simulink model "Dll_Control_AFO_V8_5_R2019b"  (R2019b)
settings: Solver=ode2  StartTime=0.0  StopTime=10  FixedStep=Ts  RelTol=1e-3
InitFcn:
  | modelDir=fileparts(get_param(bdroot,'FileName'));addpath(modelDir);rootDir=fileparts(modelDir);if isfolder(rootDir),addpath(rootDir);end;fmuDir=fullfile(rootDir,'fmu');if isfolder(fmuDir),addpath(fmuDir);end;if evalin('base','exist(''Wf0'',''var'')'),assignin('base','Wfb',evalin('base','Wf0'));end;
values from neighbouring files (symbols this model uses):
  A80 = 0.10573    [RunCtrlSysModelSHT.m]
  b11 = B(1,1)*1    [RunCtrlSysModelSHT.m]
  b21 = B(2,1)*1    [RunCtrlSysModelSHT.m]
  d31 = D(3,1)    [RunCtrlSysModelSHT.m]
  d41 = D(4,1)    [RunCtrlSysModelSHT.m]
  ExternalSecondaryAirEnabled = 0    [RunCtrlSysModelSHT.m]
  InitAir = zeros(50,1)    [RunCtrlSysModelSHT.m]
  Mkg0 = 0    [RunCtrlSysModelSHT.m]
  MkpDirectCommand = Mkp0    (= 999.278795578)    [RunCtrlSysModelSHT.m]
  MkpMax = 1200    [RunCtrlSysModelSHT.m]
  Ng0 = 38000    [RunCtrlSysModelSHT.m]
  NgMax = Ng0*1.05    (= 39900)    [RunCtrlSysModelSHT.m]
  Np0 = 20800    [RunCtrlSysModelSHT.m]
  NpDem = Np0    (= 20800)    [RunCtrlSysModelSHT.m]
  omega_u = 20    [RunCtrlSysModelSHT.m]
  power0 = 2176600    [RunCtrlSysModelSHT.m]
  RotorLoadCfg = struct(      'designNpRpm', Np0,      'designPowerW', power0,      'thetaZeroDeg', 0,      'thetaDesignDeg', 12,      'profileTorqueFraction', 0.15,      'thetaValidRangeDeg', [6, 14])    [RunCtrlSysModelSHT.m]
  RotorLoadInputMode = 'legacyPower'    [RunCtrlSysModelSHT.m]
  T45Max = 1400    [RunCtrlSysModelSHT.m]
  ThetaCommandDeg = RotorLoadCfg.thetaDesignDeg    [RunCtrlSysModelSHT.m]
  Ts = 0.025    [RunCtrlSysModelSHT.m]
  Wf0 = 0.151914044493225    (= 0.151914044493)    [RunCtrlSysModelSHT.m]
  WfMax = Wf0*2    (= 0.303828088986)    [RunCtrlSysModelSHT.m]
  WfMin = Wf0*0.01    (= 0.00151914044493)    [RunCtrlSysModelSHT.m]
  WfRateLim = 1.5    [RunCtrlSysModelSHT.m]
undefined symbols (not defined in the file or in its folder): sigbuilder_block, Wfb
libraries: simulink x10
(part 2 of 4)

== system Dll_Control_AFO_V8_5_R2019b/空气系统代理模型/G05_动力涡轮一级叶根进口 ==
  BoundaryTP24 : Inport  PortDimensions=24
  RotorSpeed_rpm : Inport  Port=2  PortDimensions=1
  GlobalParams7 : Inport  Port=3  PortDimensions=7
  EffectiveAreaScale : Selector  InputPortWidth=7  IndexOptions=Index vector (dialog)  Indices=1  OutputSizes=1
  SealCorrection : Selector  InputPortWidth=7  IndexOptions=Index vector (dialog)  Indices=7  OutputSizes=1
  可压缩节流孔口 : Subsystem  Description=Embedded ideal-gas compressible restrictor with critical pressure ratio. No external MATLAB runtime function.  mask{UpstreamBoundary=11, DownstreamBoundary=8}
      mask prompts: UpstreamBoundary "Upstream boundary index"; DownstreamBoundary "Downstream boundary index"
  导叶冷却 : Gain  Gain=0.90000000000000002
  旋转离心压升 : Subsystem  Description=Embedded centrifugal pressure rise: 0.5*kRot*rho*omega^2*(rOut^2-rIn^2).  mask{UpstreamBoundary=11, DownstreamBoundary=8}
      mask prompts: UpstreamBoundary "Upstream boundary index"; DownstreamBoundary "Downstream boundary index"
  流路可调参数 : Subsystem  Description=流路级可调物理参数（已内置在 SLX）。
  流量物理限幅 : Saturate  UpperLimit=2  LowerLimit=0
  盘腔热动态 : Subsystem  Description=Embedded discrete first-order lag with exact bypass when tau is zero.  mask{SampleTime_s=0.025000000000000001, InitialFlowValue=0.038254988453198698}
      mask prompts: SampleTime_s "Sample time [s]"; InitialFlowValue "Initial output [kg/s]"
  等效面积缩放 : Product  Inputs=**
  篦齿修正 : Product  Inputs=**
  辨识等效面积 : Subsystem  Description=辨识得到的等效面积律（内嵌 MATLAB Function）。
  G05_PT1_IN_ROOT_W_kgps : Outport
  wires:
  流量物理限幅/1 -> G05_PT1_IN_ROOT_W_kgps/1
  盘腔热动态/1(W_out) -> 流量物理限幅/1
  篦齿修正/1 -> 盘腔热动态/1(W_in)
  EffectiveAreaScale/1 -> 等效面积缩放/2
  SealCorrection/1 -> 篦齿修正/2
  导叶冷却/1 -> 篦齿修正/1
  旋转离心压升/1(W_out) -> 导叶冷却/1
  RotorSpeed_rpm/1 -> 旋转离心压升/3(RotorSpeed_rpm)
  可压缩节流孔口/1(W_kgps) -> 旋转离心压升/1(W_in)
  GlobalParams7/1 -> 可压缩节流孔口/3(GlobalParams7), 旋转离心压升/4(GlobalParams7)
  等效面积缩放/1 -> 可压缩节流孔口/2(EffectiveArea_m2)
  辨识等效面积/1(EffectiveArea_m2) -> 等效面积缩放/1
  BoundaryTP24/1 -> 可压缩节流孔口/1(BoundaryTP24), 旋转离心压升/2(BoundaryTP24), 辨识等效面积/1(BoundaryTP24)
  流路可调参数/1(RouteParams7) -> SealCorrection/1, 盘腔热动态/2(RouteParams7), 旋转离心压升/5(RouteParams7), EffectiveAreaScale/1

== system Dll_Control_AFO_V8_5_R2019b/空气系统代理模型/G06_动力涡轮一级叶根出口 ==
  BoundaryTP24 : Inport  PortDimensions=24
  RotorSpeed_rpm : Inport  Port=2  PortDimensions=1
  GlobalParams7 : Inport  Port=3  PortDimensions=7
  EffectiveAreaScale : Selector  InputPortWidth=7  IndexOptions=Index vector (dialog)  Indices=1  OutputSizes=1
  SealCorrection : Selector  InputPortWidth=7  IndexOptions=Index vector (dialog)  Indices=7  OutputSizes=1
  可压缩节流孔口 : Subsystem  Description=Embedded ideal-gas compressible restrictor with critical pressure ratio. No external MATLAB runtime function.  mask{UpstreamBoundary=11, DownstreamBoundary=5}
      mask prompts: UpstreamBoundary "Upstream boundary index"; DownstreamBoundary "Downstream boundary index"
  旋转离心压升 : Subsystem  Description=Embedded centrifugal pressure rise: 0.5*kRot*rho*omega^2*(rOut^2-rIn^2).  mask{UpstreamBoundary=11, DownstreamBoundary=5}
      mask prompts: UpstreamBoundary "Upstream boundary index"; DownstreamBoundary "Downstream boundary index"
  流路可调参数 : Subsystem  Description=流路级可调物理参数（已内置在 SLX）。
  流量物理限幅 : Saturate  UpperLimit=2  LowerLimit=0
  盘腔热动态 : Subsystem  Description=Embedded discrete first-order lag with exact bypass when tau is zero.  mask{SampleTime_s=0.025000000000000001, InitialFlowValue=0.0308724468218796}
      mask prompts: SampleTime_s "Sample time [s]"; InitialFlowValue "Initial output [kg/s]"
  等效面积缩放 : Product  Inputs=**
  篦齿修正 : Product  Inputs=**
  篦齿封严 : Gain  Gain=0.88
  辨识等效面积 : Subsystem  Description=辨识得到的等效面积律（内嵌 MATLAB Function）。
  G06_PT1_OUT_ROOT_W_kgps : Outport
  wires:
  流量物理限幅/1 -> G06_PT1_OUT_ROOT_W_kgps/1
  盘腔热动态/1(W_out) -> 流量物理限幅/1
  BoundaryTP24/1 -> 可压缩节流孔口/1(BoundaryTP24), 旋转离心压升/2(BoundaryTP24), 辨识等效面积/1(BoundaryTP24)
  篦齿修正/1 -> 盘腔热动态/1(W_in)
  EffectiveAreaScale/1 -> 等效面积缩放/2
  SealCorrection/1 -> 篦齿修正/2
  篦齿封严/1 -> 篦齿修正/1
  RotorSpeed_rpm/1 -> 旋转离心压升/3(RotorSpeed_rpm)
  旋转离心压升/1(W_out) -> 篦齿封严/1
  可压缩节流孔口/1(W_kgps) -> 旋转离心压升/1(W_in)
  辨识等效面积/1(EffectiveArea_m2) -> 等效面积缩放/1
  等效面积缩放/1 -> 可压缩节流孔口/2(EffectiveArea_m2)
  GlobalParams7/1 -> 可压缩节流孔口/3(GlobalParams7), 旋转离心压升/4(GlobalParams7)
  流路可调参数/1(RouteParams7) -> SealCorrection/1, 盘腔热动态/2(RouteParams7), 旋转离心压升/5(RouteParams7), EffectiveAreaScale/1

== system Dll_Control_AFO_V8_5_R2019b/空气系统代理模型/G07_动力涡轮二级叶尖进口 ==
  BoundaryTP24 : Inport  PortDimensions=24
  RotorSpeed_rpm : Inport  Port=2  PortDimensions=1
  GlobalParams7 : Inport  Port=3  PortDimensions=7
  EffectiveAreaScale : Selector  InputPortWidth=7  IndexOptions=Index vector (dialog)  Indices=1  OutputSizes=1
  SealCorrection : Selector  InputPortWidth=7  IndexOptions=Index vector (dialog)  Indices=7  OutputSizes=1
  可压缩节流孔口 : Subsystem  Description=Embedded ideal-gas compressible restrictor with critical pressure ratio. No external MATLAB runtime function.  mask{UpstreamBoundary=6, DownstreamBoundary=8}
      mask prompts: UpstreamBoundary "Upstream boundary index"; DownstreamBoundary "Downstream boundary index"
  旋转离心压升 : Subsystem  Description=Embedded centrifugal pressure rise: 0.5*kRot*rho*omega^2*(rOut^2-rIn^2).  mask{UpstreamBoundary=6, DownstreamBoundary=8}
      mask prompts: UpstreamBoundary "Upstream boundary index"; DownstreamBoundary "Downstream boundary index"
  流路可调参数 : Subsystem  Description=流路级可调物理参数（已内置在 SLX）。
  流量物理限幅 : Saturate  UpperLimit=2  LowerLimit=0
  盘腔热动态 : Subsystem  Description=Embedded discrete first-order lag with exact bypass when tau is zero.  mask{SampleTime_s=0.025000000000000001, InitialFlowValue=0.042952969491310798}
      mask prompts: SampleTime_s "Sample time [s]"; InitialFlowValue "Initial output [kg/s]"
  等效面积缩放 : Product  Inputs=**
  篦齿修正 : Product  Inputs=**
  篦齿封严 : Gain  Gain=0.88
  辨识等效面积 : Subsystem  Description=辨识得到的等效面积律（内嵌 MATLAB Function）。
  G07_PT2_IN_TIP_W_kgps : Outport
  wires:
  流量物理限幅/1 -> G07_PT2_IN_TIP_W_kgps/1
  盘腔热动态/1(W_out) -> 流量物理限幅/1
  流路可调参数/1(RouteParams7) -> SealCorrection/1, 盘腔热动态/2(RouteParams7), 旋转离心压升/5(RouteParams7), EffectiveAreaScale/1
  篦齿修正/1 -> 盘腔热动态/1(W_in)
  SealCorrection/1 -> 篦齿修正/2
  篦齿封严/1 -> 篦齿修正/1
  旋转离心压升/1(W_out) -> 篦齿封严/1
  可压缩节流孔口/1(W_kgps) -> 旋转离心压升/1(W_in)
  RotorSpeed_rpm/1 -> 旋转离心压升/3(RotorSpeed_rpm)
  GlobalParams7/1 -> 可压缩节流孔口/3(GlobalParams7), 旋转离心压升/4(GlobalParams7)
  等效面积缩放/1 -> 可压缩节流孔口/2(EffectiveArea_m2)
  辨识等效面积/1(EffectiveArea_m2) -> 等效面积缩放/1
  EffectiveAreaScale/1 -> 等效面积缩放/2
  BoundaryTP24/1 -> 可压缩节流孔口/1(BoundaryTP24), 旋转离心压升/2(BoundaryTP24), 辨识等效面积/1(BoundaryTP24)

== system Dll_Control_AFO_V8_5_R2019b/空气系统代理模型/G08_动力涡轮二级叶尖出口 ==
  BoundaryTP24 : Inport  PortDimensions=24
  RotorSpeed_rpm : Inport  Port=2  PortDimensions=1
  GlobalParams7 : Inport  Port=3  PortDimensions=7
  EffectiveAreaScale : Selector  InputPortWidth=7  IndexOptions=Index vector (dialog)  Indices=1  OutputSizes=1
  SealCorrection : Selector  InputPortWidth=7  IndexOptions=Index vector (dialog)  Indices=7  OutputSizes=1
  可压缩节流孔口 : Subsystem  Description=Embedded ideal-gas compressible restrictor with critical pressure ratio. No external MATLAB runtime function.  mask{UpstreamBoundary=6, DownstreamBoundary=7}
      mask prompts: UpstreamBoundary "Upstream boundary index"; DownstreamBoundary "Downstream boundary index"
  旋转离心压升 : Subsystem  Description=Embedded centrifugal pressure rise: 0.5*kRot*rho*omega^2*(rOut^2-rIn^2).  mask{UpstreamBoundary=6, DownstreamBoundary=7}
      mask prompts: UpstreamBoundary "Upstream boundary index"; DownstreamBoundary "Downstream boundary index"
  机匣冷却 : Gain  Gain=0.92000000000000004
  流路可调参数 : Subsystem  Description=流路级可调物理参数（已内置在 SLX）。
  流量物理限幅 : Saturate  UpperLimit=2  LowerLimit=0
  盘腔热动态 : Subsystem  Description=Embedded discrete first-order lag with exact bypass when tau is zero.  mask{SampleTime_s=0.025000000000000001, InitialFlowValue=0.030201306673577899}
      mask prompts: SampleTime_s "Sample time [s]"; InitialFlowValue "Initial output [kg/s]"
  等效面积缩放 : Product  Inputs=**
  篦齿修正 : Product  Inputs=**
  篦齿封严 : Gain  Gain=0.88
  辨识等效面积 : Subsystem  Description=辨识得到的等效面积律（内嵌 MATLAB Function）。
  G08_PT2_OUT_TIP_W_kgps : Outport
  wires:
  流量物理限幅/1 -> G08_PT2_OUT_TIP_W_kgps/1
  盘腔热动态/1(W_out) -> 流量物理限幅/1
  篦齿修正/1 -> 盘腔热动态/1(W_in)
  SealCorrection/1 -> 篦齿修正/2
  旋转离心压升/1(W_out) -> 机匣冷却/1
  篦齿封严/1 -> 篦齿修正/1
  机匣冷却/1 -> 篦齿封严/1
  可压缩节流孔口/1(W_kgps) -> 旋转离心压升/1(W_in)
  RotorSpeed_rpm/1 -> 旋转离心压升/3(RotorSpeed_rpm)
  GlobalParams7/1 -> 可压缩节流孔口/3(GlobalParams7), 旋转离心压升/4(GlobalParams7)
  等效面积缩放/1 -> 可压缩节流孔口/2(EffectiveArea_m2)
  辨识等效面积/1(EffectiveArea_m2) -> 等效面积缩放/1
  EffectiveAreaScale/1 -> 等效面积缩放/2
  BoundaryTP24/1 -> 可压缩节流孔口/1(BoundaryTP24), 旋转离心压升/2(BoundaryTP24), 辨识等效面积/1(BoundaryTP24)
  流路可调参数/1(RouteParams7) -> SealCorrection/1, 盘腔热动态/2(RouteParams7), 旋转离心压升/5(RouteParams7), EffectiveAreaScale/1

== system Dll_Control_AFO_V8_5_R2019b/空气系统代理模型/全局保护参数 ==
  Mux_GlobalParams7 : Mux  Inputs=7
  临界流开关 : Constant
  最低压力_Pa : Constant  Value=1000
  最低温度_K : Constant  Value=200
  最大流量_kgps : Constant  Value=2
  最小压差_Pa : Constant  Value=10
  比热比_gamma : Constant  Value=1.3999999999999999
  气体常数_JpkgK : Constant  Value=287.05000000000001
  GlobalParams7 : Outport
  wires:
  最低温度_K/1 -> Mux_GlobalParams7/1
  最低压力_Pa/1 -> Mux_GlobalParams7/2
  最小压差_Pa/1 -> Mux_GlobalParams7/3
  比热比_gamma/1 -> Mux_GlobalParams7/4
  气体常数_JpkgK/1 -> Mux_GlobalParams7/5
  最大流量_kgps/1 -> Mux_GlobalParams7/6
  临界流开关/1 -> Mux_GlobalParams7/7
  Mux_GlobalParams7/1 -> GlobalParams7/1

== system Dll_Control_AFO_V8_5_R2019b/空气系统代理模型/截面输入展开 ==
  T251_K : Inport  PortDimensions=1
  P251_Pa : Inport  Port=2  PortDimensions=1
  T252_K : Inport  Port=3  PortDimensions=1
  P252_Pa : Inport  Port=4  PortDimensions=1
  T3_K : Inport  Port=5  PortDimensions=1
  P3_Pa : Inport  Port=6  PortDimensions=1
  T4_K : Inport  Port=7  PortDimensions=1
  P4_Pa : Inport  Port=8  PortDimensions=1
  T45_K : Inport  Port=9  PortDimensions=1
  P51_Pa : Inport  Port=10  PortDimensions=1
  T5_K : Inport  Port=11  PortDimensions=1
  P45_Pa : Inport  Port=12  PortDimensions=1
  AvgP45P5 : Sum
  AvgP4P45 : Sum
  AvgT45T5 : Sum
  AvgT4T45 : Sum
  HalfP45P5 : Gain  Gain=0.5
  HalfP4P45 : Gain  Gain=0.5
  HalfT45T5 : Gain  Gain=0.5
  HalfT4T45 : Gain  Gain=0.5
  Mux_BoundaryTP24 : Mux  Inputs=24
  BoundaryTP24 : Outport
  wires:
  HalfT45T5/1 -> Mux_BoundaryTP24/15
  HalfT4T45/1 -> Mux_BoundaryTP24/17
  Mux_BoundaryTP24/1 -> BoundaryTP24/1
  P252_Pa/1 -> Mux_BoundaryTP24/22
  T252_K/1 -> Mux_BoundaryTP24/21
  P251_Pa/1 -> Mux_BoundaryTP24/12
  HalfP4P45/1 -> Mux_BoundaryTP24/18
  HalfP45P5/1 -> Mux_BoundaryTP24/16
  T251_K/1 -> Mux_BoundaryTP24/11
  AvgP4P45/1 -> HalfP4P45/1
  AvgT4T45/1 -> HalfT4T45/1
  AvgP45P5/1 -> HalfP45P5/1
  AvgT45T5/1 -> HalfT45T5/1
  P3_Pa/1 -> Mux_BoundaryTP24/20, Mux_BoundaryTP24/24
  T3_K/1 -> Mux_BoundaryTP24/19, Mux_BoundaryTP24/23
  P4_Pa/1 -> Mux_BoundaryTP24/4, Mux_BoundaryTP24/8, Mux_BoundaryTP24/6, AvgP4P45/1
  T4_K/1 -> Mux_BoundaryTP24/5, Mux_BoundaryTP24/7, Mux_BoundaryTP24/3, AvgT4T45/1
  P45_Pa/1 -> AvgP45P5/2, Mux_BoundaryTP24/10
  P51_Pa/1 -> Mux_BoundaryTP24/2, Mux_BoundaryTP24/14, AvgP4P45/2, AvgP45P5/1
  T5_K/1 -> AvgT45T5/2, Mux_BoundaryTP24/9
  T45_K/1 -> Mux_BoundaryTP24/1, AvgT45T5/1, Mux_BoundaryTP24/13, AvgT4T45/2

== system Dll_Control_AFO_V8_5_R2019b/滑油系统代理模型/滑油系统代理核心/支路_流量压力分配 ==
  note: ② A/B 轴承腔供油与回油
  note: ③ 散热器耦合边界
  输入向量 : Inport
  kRet_A : Gain  Gain=0.96
  kRet_B : Gain  Gain=0.96
  核心流量压力计算 : Subsystem
  甲轴承腔流量 : Outport
  乙轴承腔流量 : Outport  Port=2
  甲轴承腔压力 : Outport  Port=3
  乙轴承腔压力 : Outport  Port=4
  A腔回油流量 : Outport  Port=5
  B腔回油流量 : Outport  Port=6
  QG_m3_s : Outport  Port=7
  Pman_Pa : Outport  Port=8
  Pret_Pa : Outport  Port=9
  wires:
  输入向量/1 -> 核心流量压力计算/1(u26)  "u26"
  核心流量压力计算/1(QA_m3_s) -> 甲轴承腔流量/1, kRet_A/1  "QA_m3_s"
  kRet_A/1 -> A腔回油流量/1  "QretA_m3_s"
  核心流量压力计算/2(QB_m3_s) -> 乙轴承腔流量/1, kRet_B/1  "QB_m3_s"
  kRet_B/1 -> B腔回油流量/1  "QretB_m3_s"
  核心流量压力计算/3(PA_Pa) -> 甲轴承腔压力/1  "PA_Pa"
  核心流量压力计算/4(PB_Pa) -> 乙轴承腔压力/1  "PB_Pa"
  核心流量压力计算/5(QG_m3_s) -> QG_m3_s/1  "QG_m3_s"
  核心流量压力计算/6(Pman_Pa) -> Pman_Pa/1  "Pman_Pa"
  核心流量压力计算/7(Pret_Pa) -> Pret_Pa/1  "Pret_Pa"

== system Dll_Control_AFO_V8_5_R2019b/滑油系统代理模型/滑油系统代理核心/支路_燃滑散热 ==
  输入向量 : Inport
  QA_m3_s : Inport  Port=2
  QB_m3_s : Inport  Port=3
  QG_m3_s : Inport  Port=4
  Pman_Pa : Inport  Port=5
  PA_Pa : Inport  Port=6
  PB_Pa : Inport  Port=7
  Abs_Wfuel : Abs
  Demux_FP_Coupling : Demux  Outputs=3
  FCN_FuelOil_FP_Coupling : MATLAB Function  TreatAsAtomicUnit=on
  FuelTout_sum : Sum
  Q_raw : Product  Inputs=****
  SEL_Tfuel : Selector  InputPortWidth=26  IndexOptions=Index vector (dialog)  Indices=25  OutputSizes=1
  SEL_Toil : Selector  InputPortWidth=26  IndexOptions=Index vector (dialog)  Indices=9  OutputSizes=1
  SEL_Wfuel : Selector  InputPortWidth=26  IndexOptions=Index vector (dialog)  Indices=26  OutputSizes=1
  Sqrt_Wfuel : Math  Operator=sqrt  SignedPower=off  SaturateOnIntegerOverflow=on
  Wfuel_eps : Sum
  dT : Sum  Inputs=+-
  eps : Constant  Value=1e-3
  kTf : Gain  Gain=1.0e-4
  kUA : Gain  Gain=145
  FuelOilCooler_Q : Outport
  FuelOilCooler_FuelTout : Outport  Port=2
  FuelOilCooler_Pin_Pa : Outport  Port=3
  FuelOilCooler_Pout_Pa : Outport  Port=4
  wires:
  FCN_FuelOil_FP_Coupling/1(y) -> Demux_FP_Coupling/1
  Demux_FP_Coupling/3 -> FuelOilCooler_Pout_Pa/1
  Demux_FP_Coupling/2 -> FuelOilCooler_Pin_Pa/1
  Demux_FP_Coupling/1 -> Q_raw/4
  SEL_Wfuel/1 -> Abs_Wfuel/1
  Sqrt_Wfuel/1 -> Q_raw/2
  FuelTout_sum/1 -> FuelOilCooler_FuelTout/1
  dT/1 -> Q_raw/1
  Wfuel_eps/1 -> Sqrt_Wfuel/1
  SEL_Toil/1 -> dT/1
  kTf/1 -> FuelTout_sum/2
  Q_raw/1 -> kUA/1
  Abs_Wfuel/1 -> Wfuel_eps/1
  eps/1 -> Wfuel_eps/2, Q_raw/3
  输入向量/1 -> SEL_Toil/1, SEL_Wfuel/1, SEL_Tfuel/1
  kUA/1 -> FuelOilCooler_Q/1, kTf/1
  SEL_Tfuel/1 -> dT/2, FuelTout_sum/1
  QA_m3_s/1 -> FCN_FuelOil_FP_Coupling/1(QA)
  QB_m3_s/1 -> FCN_FuelOil_FP_Coupling/2(QB)
  QG_m3_s/1 -> FCN_FuelOil_FP_Coupling/3(QG)
  Pman_Pa/1 -> FCN_FuelOil_FP_Coupling/4(Pman)
  PA_Pa/1 -> FCN_FuelOil_FP_Coupling/5(PA)
  PB_Pa/1 -> FCN_FuelOil_FP_Coupling/6(PB)

== system Dll_Control_AFO_V8_5_R2019b/滑油系统代理模型/滑油系统代理核心/支路_空滑换热 ==
  输入向量 : Inport
  QretA_m3_s : Inport  Port=2
  QretB_m3_s : Inport  Port=3
  Pret_Pa : Inport  Port=4
  FCN_AOH_Formula : MATLAB Function  TreatAsAtomicUnit=on
  FCN_AOH_Predict : MATLAB Function  TreatAsAtomicUnit=on
  SEL_IN_01 : Selector  InputPortWidth=26  IndexOptions=Index vector (dialog)  Indices=9  OutputSizes=1
  关键输入监视终端 : Terminator
  关键输入缩放 : Gain  Gain=0.1
  输出拆分 : Demux  Outputs=3
  输出融合 : Sum
  空滑换热量 : Outport
  AirOilCooler_Pin_Pa : Outport  Port=2
  AirOilCooler_Pout_Pa : Outport  Port=3
  wires:
  关键输入缩放/1 -> 关键输入监视终端/1
  输出拆分/2 -> AirOilCooler_Pin_Pa/1
  输出拆分/3 -> AirOilCooler_Pout_Pa/1
  SEL_IN_01/1 -> 关键输入缩放/1
  QretA_m3_s/1 -> FCN_AOH_Formula/2(QretA)
  FCN_AOH_Predict/1(y) -> 输出融合/1
  输出拆分/1 -> 空滑换热量/1
  FCN_AOH_Formula/1(y) -> 输出融合/2
  输出融合/1 -> 输出拆分/1
  输入向量/1 -> FCN_AOH_Predict/1(u), FCN_AOH_Formula/1(u), SEL_IN_01/1
  QretB_m3_s/1 -> FCN_AOH_Formula/3(QretB)
  Pret_Pa/1 -> FCN_AOH_Formula/4(Pret)

== system Dll_Control_AFO_V8_5_R2019b/滑油系统代理模型/滑油系统代理核心/支路_轴承甲乙换热 ==
  输入向量 : Inport
  A总生热 : Sum
  A换热叠加 : Sum
  A轴承N2_生热 : Math  Operator=square  SignedPower=off  SaturateOnIntegerOverflow=on
  B总生热 : Sum
  B换热叠加 : Sum
  B轴承N2_生热 : Math  Operator=square  SignedPower=off  SaturateOnIntegerOverflow=on
  FCN_BRG_Formula : MATLAB Function  TreatAsAtomicUnit=on
  FCN_BRG_Predict : MATLAB Function  TreatAsAtomicUnit=on
  SEL_IN_01 : Selector  InputPortWidth=26  IndexOptions=Index vector (dialog)  Indices=1  OutputSizes=1
  SEL_IN_02 : Selector  InputPortWidth=26  IndexOptions=Index vector (dialog)  Indices=2  OutputSizes=1
  kBrgHeat_A : Gain  Gain=1.5573407202216067e-06
  kBrgHeat_B : Gain  Gain=7.7434124676632876e-06
  kSealHeat_A : Gain  Gain=3.8933518005540168e-07
  kSealHeat_B : Gain  Gain=1.9358531169158219e-06
  输出拆分 : Demux
  输出融合 : Sum
  甲轴承腔换热量 : Outport
  乙轴承腔换热量 : Outport  Port=2
  甲轴承腔出口油温 : Outport  Port=3
  乙轴承腔出口油温 : Outport  Port=4
  甲轴承腔生热量 : Outport  Port=5
  乙轴承腔生热量 : Outport  Port=6
  wires:
  输出拆分/1 -> A换热叠加/1
  输出拆分/3 -> 甲轴承腔出口油温/1
  kSealHeat_A/1 -> A总生热/2
  输出拆分/4 -> 乙轴承腔出口油温/1
  B轴承N2_生热/1 -> kBrgHeat_B/1, kSealHeat_B/1
  输出融合/1 -> 输出拆分/1
  A轴承N2_生热/1 -> kBrgHeat_A/1, kSealHeat_A/1
  B总生热/1 -> B换热叠加/2, 乙轴承腔生热量/1
  输出拆分/2 -> B换热叠加/1
  A换热叠加/1 -> 甲轴承腔换热量/1
  SEL_IN_01/1 -> A轴承N2_生热/1
  kBrgHeat_B/1 -> B总生热/1
  kSealHeat_B/1 -> B总生热/2
  A总生热/1 -> A换热叠加/2, 甲轴承腔生热量/1
  B换热叠加/1 -> 乙轴承腔换热量/1
  kBrgHeat_A/1 -> A总生热/1
  输入向量/1 -> SEL_IN_02/1, FCN_BRG_Formula/1(u), FCN_BRG_Predict/1(u), SEL_IN_01/1
  SEL_IN_02/1 -> B轴承N2_生热/1
  FCN_BRG_Formula/1(y) -> 输出融合/2
  FCN_BRG_Predict/1(y) -> 输出融合/1

== system Dll_Control_AFO_V8_5_R2019b/滑油系统代理模型/滑油系统代理核心/支路机匣附件换热 ==
  输入向量 : Inport
  FCN_CAS_Formula : MATLAB Function  TreatAsAtomicUnit=on
  FCN_CAS_Predict : MATLAB Function  TreatAsAtomicUnit=on
  输出拆分 : Demux  Outputs=1
  输出融合 : Sum
  机匣附件换热量 : Outport
  wires:
  输入向量/1 -> FCN_CAS_Predict/1(u), FCN_CAS_Formula/1(u)
  输出融合/1 -> 输出拆分/1
  输出拆分/1 -> 机匣附件换热量/1
  FCN_CAS_Formula/1(y) -> 输出融合/2
  FCN_CAS_Predict/1(y) -> 输出融合/1

== system Dll_Control_AFO_V8_5_R2019b/燃油系统代理模型1/燃油系统代理模型/1//(0.005*s+1) ==
  uk : Inport
  u0 : Inport  Port=2
  y0 : Inport  Port=3
  Gain3 : Gain  Gain=Ts
  Gain6 : Gain  Gain=Ts
  Gain7 : Gain  Gain=0.01-Ts
  Gain8 : Gain  Gain=1/(0.01+Ts)
  Sum3 : Sum  Inputs=+++
  u_k_1 : Delay  DelayLength=1  InitialConditionSource=Input port
      settings: InputPortMap=u0,p4
  y_k_1 : Delay  DelayLength=1  InitialConditionSource=Input port
      settings: InputPortMap=u0,p4
  y : Outport
  wires:
  u0/1 -> u_k_1/2
  y0/1 -> y_k_1/2
  y_k_1/1 -> Gain7/1
  Gain3/1 -> Sum3/1
  Gain7/1 -> Sum3/3
  Gain6/1 -> Sum3/2
  uk/1 -> Gain3/1, u_k_1/1
  Gain8/1 -> y/1, y_k_1/1
  u_k_1/1 -> Gain6/1
  Sum3/1 -> Gain8/1

== system Dll_Control_AFO_V8_5_R2019b/燃油系统代理模型1/燃油系统代理模型/1//(0.005*s+1)Sys1 ==
  uk : Inport
  u0 : Inport  Port=2
  y0 : Inport  Port=3
  Gain3 : Gain  Gain=Ts
  Gain6 : Gain  Gain=Ts
  Gain7 : Gain  Gain=0.01-Ts
  Gain8 : Gain  Gain=1/(0.01+Ts)
  Sum3 : Sum  Inputs=+++
  u_k_1 : Delay  DelayLength=1  InitialConditionSource=Input port
      settings: InputPortMap=u0,p4
  y_k_1 : Delay  DelayLength=1  InitialConditionSource=Input port
      settings: InputPortMap=u0,p4
  y : Outport
  wires:
  u0/1 -> u_k_1/2
  y0/1 -> y_k_1/2
  y_k_1/1 -> Gain7/1
  Gain3/1 -> Sum3/1
  Gain7/1 -> Sum3/3
  Gain6/1 -> Sum3/2
  uk/1 -> Gain3/1, u_k_1/1
  Gain8/1 -> y/1, y_k_1/1
  u_k_1/1 -> Gain6/1
  Sum3/1 -> Gain8/1

== system Dll_Control_AFO_V8_5_R2019b/空气系统代理模型/G01_燃气涡轮一级进口/可压缩节流孔口 ==
  BoundaryTP24 : Inport  PortDimensions=24
  EffectiveArea_m2 : Inport  Port=2  PortDimensions=1
  GlobalParams7 : Inport  Port=3  PortDimensions=7
  ApplyMaximumFlow : MinMax  Inputs=2
  BoundRatio : Saturate  UpperLimit=1  LowerLimit=1e-6
  CriticalEnabled : Selector  InputPortWidth=7  IndexOptions=Index vector (dialog)  Indices=7  OutputSizes=1
  CriticalRatio : Fcn  Expr=(2/(u+1))^(u/(u-1))
  EnableForwardFlow : Switch  Criteria=u2 ~= 0
  ForwardFlow : RelationalOperator  Operator=>  OutDataTypeStr=boolean  RndMeth=Simplest
  Gamma : Selector  InputPortWidth=7  IndexOptions=Index vector (dialog)  Indices=4  OutputSizes=1
  GasR : Selector  InputPortWidth=7  IndexOptions=Index vector (dialog)  Indices=5  OutputSizes=1
  IsChoked : RelationalOperator  Operator=<=  OutDataTypeStr=boolean  RndMeth=Simplest
  MassFlowRaw : Product  Inputs=***/
  MuxGammaRatio : Mux  Inputs=2
  PhiChoked : Fcn  Expr=sqrt(u)*(2/(u+1))^((u+1)/(2*(u-1)))
  PhiSubcritical : Fcn  Expr=sqrt(2*u(1)/(u(1)-1)*(u(2)^(2/u(1))-u(2)^((u(1)+1)/u(1))))
  Pin_raw : Selector  InputPortWidth=24  IndexOptions=Index vector (dialog)  Indices=2*UpstreamBoundary  OutputSizes=1
  Pmin : Selector  InputPortWidth=7  IndexOptions=Index vector (dialog)  Indices=2  OutputSizes=1
  PoutPlusMinimumDrop : Sum
  Pout_raw : Selector  InputPortWidth=24  IndexOptions=Index vector (dialog)  Indices=2*DownstreamBoundary  OutputSizes=1
  PressureRatio : Product  Inputs=*/
  ProtectPin : MinMax  Function=max  Inputs=2
  ProtectPout : MinMax  Function=max  Inputs=2
  ProtectTin : MinMax  Function=max  Inputs=2
  RT : Product  Inputs=**
  SelectPhi : Switch  Criteria=u2 ~= 0
  SqrtRT : Math  Operator=sqrt  SignedPower=off  SaturateOnIntegerOverflow=on
  Tin_raw : Selector  InputPortWidth=24  IndexOptions=Index vector (dialog)  Indices=2*UpstreamBoundary-1  OutputSizes=1
  Tmin : Selector  InputPortWidth=7  IndexOptions=Index vector (dialog)  Indices=1  OutputSizes=1
  UseChokedBranch : Logic  AllPortsSameDT=off  OutDataTypeStr=boolean
  Wmax : Selector  InputPortWidth=7  IndexOptions=Index vector (dialog)  Indices=6  OutputSizes=1
  ZeroFlow : Constant  Value=0
  dPmin : Selector  InputPortWidth=7  IndexOptions=Index vector (dialog)  Indices=3  OutputSizes=1
  W_kgps : Outport
  wires:
  ApplyMaximumFlow/1 -> W_kgps/1
  Wmax/1 -> ApplyMaximumFlow/2
  EnableForwardFlow/1 -> ApplyMaximumFlow/1
  ZeroFlow/1 -> EnableForwardFlow/3
  ForwardFlow/1 -> EnableForwardFlow/2
  MassFlowRaw/1 -> EnableForwardFlow/1
  SqrtRT/1 -> MassFlowRaw/4
  EffectiveArea_m2/1 -> MassFlowRaw/3
  SelectPhi/1 -> MassFlowRaw/2
  RT/1 -> SqrtRT/1
  ProtectTin/1 -> RT/2
  GasR/1 -> RT/1
  PhiSubcritical/1 -> SelectPhi/3
  UseChokedBranch/1 -> SelectPhi/2
  PhiChoked/1 -> SelectPhi/1
  CriticalEnabled/1 -> UseChokedBranch/2
  IsChoked/1 -> UseChokedBranch/1
  CriticalRatio/1 -> IsChoked/2
  MuxGammaRatio/1 -> PhiSubcritical/1
  BoundRatio/1 -> IsChoked/1, MuxGammaRatio/2
  Gamma/1 -> MuxGammaRatio/1, PhiChoked/1, CriticalRatio/1
  PressureRatio/1 -> BoundRatio/1
  PoutPlusMinimumDrop/1 -> ForwardFlow/2
  ProtectPin/1 -> MassFlowRaw/1, PressureRatio/2, ForwardFlow/1
  dPmin/1 -> PoutPlusMinimumDrop/2
  ProtectPout/1 -> PressureRatio/1, PoutPlusMinimumDrop/1
  Pout_raw/1 -> ProtectPout/1
  Pmin/1 -> ProtectPout/2, ProtectPin/2
  Pin_raw/1 -> ProtectPin/1
  Tmin/1 -> ProtectTin/2
  Tin_raw/1 -> ProtectTin/1
  GlobalParams7/1 -> CriticalEnabled/1, Wmax/1, GasR/1, Gamma/1, dPmin/1, Pmin/1, Tmin/1
  BoundaryTP24/1 -> Pout_raw/1, Pin_raw/1, Tin_raw/1

== system Dll_Control_AFO_V8_5_R2019b/空气系统代理模型/G01_燃气涡轮一级进口/流路可调参数 ==
  Mux_RouteParams7 : Mux  Inputs=7
  kRot : Constant  Value=0
  内半径_m : Constant  Value=0
  初值流量_kgps : Constant  Value=0.54362352012440196
  外半径_m : Constant  Value=0
  时间常数_s : Constant  Value=0
  等效面积缩放 : Constant  Value=0.98690787759156895
  篦齿修正系数 : Constant
  RouteParams7 : Outport
  wires:
  等效面积缩放/1 -> Mux_RouteParams7/1
  kRot/1 -> Mux_RouteParams7/2
  内半径_m/1 -> Mux_RouteParams7/3
  外半径_m/1 -> Mux_RouteParams7/4
  时间常数_s/1 -> Mux_RouteParams7/5
  初值流量_kgps/1 -> Mux_RouteParams7/6
  篦齿修正系数/1 -> Mux_RouteParams7/7
  Mux_RouteParams7/1 -> RouteParams7/1

== system Dll_Control_AFO_V8_5_R2019b/空气系统代理模型/G01_燃气涡轮一级进口/盘腔热动态 ==
  W_in : Inport  PortDimensions=1
  RouteParams7 : Inport  Port=2  PortDimensions=7
  Alpha : Fcn  Expr=exp(-SampleTime_s/u)
  DynamicOrBypass : Switch  Criteria=u2 ~= 0
  One : Constant
  OneMinusAlpha : Sum  Inputs=+-
  ProtectTau : Saturate  UpperLimit=inf  LowerLimit=1e-9
  State : UnitDelay  InitialCondition=InitialFlowValue  SampleTime=SampleTime_s  HasFrameUpgradeWarning=on
  Tau_s : Selector  InputPortWidth=7  IndexOptions=Index vector (dialog)  Indices=5  OutputSizes=1
  Update : Sum
  UseBypass : simulink/Logic and Bit Operations/Compare To Constant  relop=<=  const=1e-12  OutDataTypeStr=boolean
  WeightedInput : Product  Inputs=**
  WeightedState : Product  Inputs=**
  W_out : Outport
  wires:
  DynamicOrBypass/1 -> W_out/1
  UseBypass/1 -> DynamicOrBypass/2
  Update/1 -> DynamicOrBypass/3, State/1
  WeightedState/1 -> Update/2
  WeightedInput/1 -> Update/1
  State/1 -> WeightedState/1
  OneMinusAlpha/1 -> WeightedInput/2
  W_in/1 -> DynamicOrBypass/1, WeightedInput/1
  Alpha/1 -> WeightedState/2, OneMinusAlpha/2
  One/1 -> OneMinusAlpha/1
  ProtectTau/1 -> Alpha/1
  Tau_s/1 -> UseBypass/1, ProtectTau/1
  RouteParams7/1 -> Tau_s/1

== system Dll_Control_AFO_V8_5_R2019b/空气系统代理模型/G01_燃气涡轮一级进口/辨识等效面积 ==
  BoundaryTP24 : Inport  PortDimensions=24
  IdentifiedAreaLaw : MATLAB Function  TreatAsAtomicUnit=on
  EffectiveArea_m2 : Outport
  wires:
  BoundaryTP24/1 -> IdentifiedAreaLaw/1(boundaryTP24)
  IdentifiedAreaLaw/1(area) -> EffectiveArea_m2/1

== system Dll_Control_AFO_V8_5_R2019b/空气系统代理模型/G02_燃气涡轮一级出口/可压缩节流孔口 ==
  BoundaryTP24 : Inport  PortDimensions=24
  EffectiveArea_m2 : Inport  Port=2  PortDimensions=1
  GlobalParams7 : Inport  Port=3  PortDimensions=7
  ApplyMaximumFlow : MinMax  Inputs=2
  BoundRatio : Saturate  UpperLimit=1  LowerLimit=1e-6
  CriticalEnabled : Selector  InputPortWidth=7  IndexOptions=Index vector (dialog)  Indices=7  OutputSizes=1
  CriticalRatio : Fcn  Expr=(2/(u+1))^(u/(u-1))
  EnableForwardFlow : Switch  Criteria=u2 ~= 0
  ForwardFlow : RelationalOperator  Operator=>  OutDataTypeStr=boolean  RndMeth=Simplest
  Gamma : Selector  InputPortWidth=7  IndexOptions=Index vector (dialog)  Indices=4  OutputSizes=1
  GasR : Selector  InputPortWidth=7  IndexOptions=Index vector (dialog)  Indices=5  OutputSizes=1
  IsChoked : RelationalOperator  Operator=<=  OutDataTypeStr=boolean  RndMeth=Simplest
  MassFlowRaw : Product  Inputs=***/
  MuxGammaRatio : Mux  Inputs=2
  PhiChoked : Fcn  Expr=sqrt(u)*(2/(u+1))^((u+1)/(2*(u-1)))
  PhiSubcritical : Fcn  Expr=sqrt(2*u(1)/(u(1)-1)*(u(2)^(2/u(1))-u(2)^((u(1)+1)/u(1))))
  Pin_raw : Selector  InputPortWidth=24  IndexOptions=Index vector (dialog)  Indices=2*UpstreamBoundary  OutputSizes=1
  Pmin : Selector  InputPortWidth=7  IndexOptions=Index vector (dialog)  Indices=2  OutputSizes=1
  PoutPlusMinimumDrop : Sum
  Pout_raw : Selector  InputPortWidth=24  IndexOptions=Index vector (dialog)  Indices=2*DownstreamBoundary  OutputSizes=1
  PressureRatio : Product  Inputs=*/
  ProtectPin : MinMax  Function=max  Inputs=2
  ProtectPout : MinMax  Function=max  Inputs=2
  ProtectTin : MinMax  Function=max  Inputs=2
  RT : Product  Inputs=**
  SelectPhi : Switch  Criteria=u2 ~= 0
  SqrtRT : Math  Operator=sqrt  SignedPower=off  SaturateOnIntegerOverflow=on
  Tin_raw : Selector  InputPortWidth=24  IndexOptions=Index vector (dialog)  Indices=2*UpstreamBoundary-1  OutputSizes=1
  Tmin : Selector  InputPortWidth=7  IndexOptions=Index vector (dialog)  Indices=1  OutputSizes=1
  UseChokedBranch : Logic  AllPortsSameDT=off  OutDataTypeStr=boolean
  Wmax : Selector  InputPortWidth=7  IndexOptions=Index vector (dialog)  Indices=6  OutputSizes=1
  ZeroFlow : Constant  Value=0
  dPmin : Selector  InputPortWidth=7  IndexOptions=Index vector (dialog)  Indices=3  OutputSizes=1
  W_kgps : Outport
  wires:
  ApplyMaximumFlow/1 -> W_kgps/1
  Wmax/1 -> ApplyMaximumFlow/2
  EnableForwardFlow/1 -> ApplyMaximumFlow/1
  ZeroFlow/1 -> EnableForwardFlow/3
  ForwardFlow/1 -> EnableForwardFlow/2
  MassFlowRaw/1 -> EnableForwardFlow/1
  SqrtRT/1 -> MassFlowRaw/4
  EffectiveArea_m2/1 -> MassFlowRaw/3
  SelectPhi/1 -> MassFlowRaw/2
  RT/1 -> SqrtRT/1
  ProtectTin/1 -> RT/2
  GasR/1 -> RT/1
  PhiSubcritical/1 -> SelectPhi/3
  UseChokedBranch/1 -> SelectPhi/2
  PhiChoked/1 -> SelectPhi/1
  CriticalEnabled/1 -> UseChokedBranch/2
  IsChoked/1 -> UseChokedBranch/1
  CriticalRatio/1 -> IsChoked/2
  MuxGammaRatio/1 -> PhiSubcritical/1
  BoundRatio/1 -> IsChoked/1, MuxGammaRatio/2
  Gamma/1 -> MuxGammaRatio/1, PhiChoked/1, CriticalRatio/1
  PressureRatio/1 -> BoundRatio/1
  PoutPlusMinimumDrop/1 -> ForwardFlow/2
  ProtectPin/1 -> MassFlowRaw/1, PressureRatio/2, ForwardFlow/1
  dPmin/1 -> PoutPlusMinimumDrop/2
  ProtectPout/1 -> PressureRatio/1, PoutPlusMinimumDrop/1
  Pout_raw/1 -> ProtectPout/1
  Pmin/1 -> ProtectPout/2, ProtectPin/2
  Pin_raw/1 -> ProtectPin/1
  Tmin/1 -> ProtectTin/2
  Tin_raw/1 -> ProtectTin/1
  GlobalParams7/1 -> CriticalEnabled/1, Wmax/1, GasR/1, Gamma/1, dPmin/1, Pmin/1, Tmin/1
  BoundaryTP24/1 -> Pout_raw/1, Pin_raw/1, Tin_raw/1

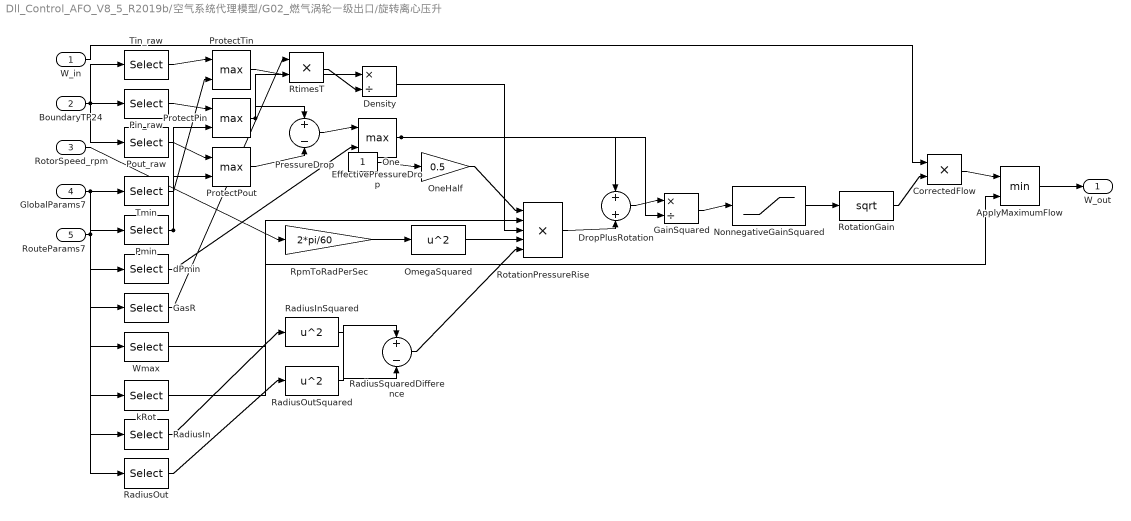
== system Dll_Control_AFO_V8_5_R2019b/空气系统代理模型/G02_燃气涡轮一级出口/旋转离心压升 ==
  W_in : Inport  PortDimensions=1
  BoundaryTP24 : Inport  Port=2  PortDimensions=24
  RotorSpeed_rpm : Inport  Port=3  PortDimensions=1
  GlobalParams7 : Inport  Port=4  PortDimensions=7
  RouteParams7 : Inport  Port=5  PortDimensions=7
  ApplyMaximumFlow : MinMax  Inputs=2
  CorrectedFlow : Product  Inputs=**
  Density : Product  Inputs=*/
  DropPlusRotation : Sum
  EffectivePressureDrop : MinMax  Function=max  Inputs=2
  GainSquared : Product  Inputs=*/
  GasR : Selector  InputPortWidth=7  IndexOptions=Index vector (dialog)  Indices=5  OutputSizes=1
  NonnegativeGainSquared : Saturate  UpperLimit=16  LowerLimit=0
  OmegaSquared : Math  Operator=square  SignedPower=off  SaturateOnIntegerOverflow=on
  One : Constant
  OneHalf : Gain  Gain=0.5
  Pin_raw : Selector  InputPortWidth=24  IndexOptions=Index vector (dialog)  Indices=2*UpstreamBoundary  OutputSizes=1
  Pmin : Selector  InputPortWidth=7  IndexOptions=Index vector (dialog)  Indices=2  OutputSizes=1
  Pout_raw : Selector  InputPortWidth=24  IndexOptions=Index vector (dialog)  Indices=2*DownstreamBoundary  OutputSizes=1
  PressureDrop : Sum  Inputs=+-
  ProtectPin : MinMax  Function=max  Inputs=2
  ProtectPout : MinMax  Function=max  Inputs=2
  ProtectTin : MinMax  Function=max  Inputs=2
  RadiusIn : Selector  InputPortWidth=7  IndexOptions=Index vector (dialog)  Indices=3  OutputSizes=1
  RadiusInSquared : Math  Operator=square  SignedPower=off  SaturateOnIntegerOverflow=on
  RadiusOut : Selector  InputPortWidth=7  IndexOptions=Index vector (dialog)  Indices=4  OutputSizes=1
  RadiusOutSquared : Math  Operator=square  SignedPower=off  SaturateOnIntegerOverflow=on
  RadiusSquaredDifference : Sum  Inputs=+-
  RotationGain : Math  Operator=sqrt  SignedPower=off  SaturateOnIntegerOverflow=on
  RotationPressureRise : Product  Inputs=*****
  RpmToRadPerSec : Gain  Gain=2*pi/60
  RtimesT : Product  Inputs=**
  Tin_raw : Selector  InputPortWidth=24  IndexOptions=Index vector (dialog)  Indices=2*UpstreamBoundary-1  OutputSizes=1
  Tmin : Selector  InputPortWidth=7  IndexOptions=Index vector (dialog)  Indices=1  OutputSizes=1
  Wmax : Selector  InputPortWidth=7  IndexOptions=Index vector (dialog)  Indices=6  OutputSizes=1
  dPmin : Selector  InputPortWidth=7  IndexOptions=Index vector (dialog)  Indices=3  OutputSizes=1
  kRot : Selector  InputPortWidth=7  IndexOptions=Index vector (dialog)  Indices=2  OutputSizes=1
  W_out : Outport
  wires:
  ApplyMaximumFlow/1 -> W_out/1
  Wmax/1 -> ApplyMaximumFlow/2
  CorrectedFlow/1 -> ApplyMaximumFlow/1
  RotationGain/1 -> CorrectedFlow/2
  W_in/1 -> CorrectedFlow/1
  NonnegativeGainSquared/1 -> RotationGain/1
  GainSquared/1 -> NonnegativeGainSquared/1
  DropPlusRotation/1 -> GainSquared/1
  RotationPressureRise/1 -> DropPlusRotation/2
  EffectivePressureDrop/1 -> GainSquared/2, DropPlusRotation/1
  dPmin/1 -> EffectivePressureDrop/2
  PressureDrop/1 -> EffectivePressureDrop/1
  ProtectPout/1 -> PressureDrop/2
  RadiusSquaredDifference/1 -> RotationPressureRise/5
  OmegaSquared/1 -> RotationPressureRise/4
  Density/1 -> RotationPressureRise/3
  kRot/1 -> RotationPressureRise/2
  OneHalf/1 -> RotationPressureRise/1
  One/1 -> OneHalf/1
  RadiusInSquared/1 -> RadiusSquaredDifference/2
  RadiusOutSquared/1 -> RadiusSquaredDifference/1
  RadiusOut/1 -> RadiusOutSquared/1
  RadiusIn/1 -> RadiusInSquared/1
  RpmToRadPerSec/1 -> OmegaSquared/1
  RotorSpeed_rpm/1 -> RpmToRadPerSec/1
  RtimesT/1 -> Density/2
  ProtectPin/1 -> PressureDrop/1, Density/1
  ProtectTin/1 -> RtimesT/2
  GasR/1 -> RtimesT/1
  Pout_raw/1 -> ProtectPout/1
  Pmin/1 -> ProtectPout/2, ProtectPin/2
  Pin_raw/1 -> ProtectPin/1
  Tmin/1 -> ProtectTin/2
  Tin_raw/1 -> ProtectTin/1
  RouteParams7/1 -> RadiusOut/1, RadiusIn/1, kRot/1
  GlobalParams7/1 -> Wmax/1, GasR/1, dPmin/1, Pmin/1, Tmin/1
  BoundaryTP24/1 -> Pout_raw/1, Pin_raw/1, Tin_raw/1

== system Dll_Control_AFO_V8_5_R2019b/空气系统代理模型/G02_燃气涡轮一级出口/流路可调参数 ==
  Mux_RouteParams7 : Mux  Inputs=7
  kRot : Constant  Value=0.5
  内半径_m : Constant  Value=0.029899999999999999
  初值流量_kgps : Constant  Value=0.20536888538032999
  外半径_m : Constant  Value=0.031300000000000001
  时间常数_s : Constant  Value=0
  等效面积缩放 : Constant  Value=0.98688005042097871
  篦齿修正系数 : Constant
  RouteParams7 : Outport
  wires:
  等效面积缩放/1 -> Mux_RouteParams7/1
  kRot/1 -> Mux_RouteParams7/2
  内半径_m/1 -> Mux_RouteParams7/3
  外半径_m/1 -> Mux_RouteParams7/4
  时间常数_s/1 -> Mux_RouteParams7/5
  初值流量_kgps/1 -> Mux_RouteParams7/6
  篦齿修正系数/1 -> Mux_RouteParams7/7
  Mux_RouteParams7/1 -> RouteParams7/1

== system Dll_Control_AFO_V8_5_R2019b/空气系统代理模型/G02_燃气涡轮一级出口/盘腔热动态 ==
  W_in : Inport  PortDimensions=1
  RouteParams7 : Inport  Port=2  PortDimensions=7
  Alpha : Fcn  Expr=exp(-SampleTime_s/u)
  DynamicOrBypass : Switch  Criteria=u2 ~= 0
  One : Constant
  OneMinusAlpha : Sum  Inputs=+-
  ProtectTau : Saturate  UpperLimit=inf  LowerLimit=1e-9
  State : UnitDelay  InitialCondition=InitialFlowValue  SampleTime=SampleTime_s  HasFrameUpgradeWarning=on
  Tau_s : Selector  InputPortWidth=7  IndexOptions=Index vector (dialog)  Indices=5  OutputSizes=1
  Update : Sum
  UseBypass : simulink/Logic and Bit Operations/Compare To Constant  relop=<=  const=1e-12  OutDataTypeStr=boolean
  WeightedInput : Product  Inputs=**
  WeightedState : Product  Inputs=**
  W_out : Outport
  wires:
  DynamicOrBypass/1 -> W_out/1
  UseBypass/1 -> DynamicOrBypass/2
  Update/1 -> DynamicOrBypass/3, State/1
  WeightedState/1 -> Update/2
  WeightedInput/1 -> Update/1
  State/1 -> WeightedState/1
  OneMinusAlpha/1 -> WeightedInput/2
  W_in/1 -> DynamicOrBypass/1, WeightedInput/1
  Alpha/1 -> WeightedState/2, OneMinusAlpha/2
  One/1 -> OneMinusAlpha/1
  ProtectTau/1 -> Alpha/1
  Tau_s/1 -> UseBypass/1, ProtectTau/1
  RouteParams7/1 -> Tau_s/1

== system Dll_Control_AFO_V8_5_R2019b/空气系统代理模型/G02_燃气涡轮一级出口/辨识等效面积 ==
  BoundaryTP24 : Inport  PortDimensions=24
  IdentifiedAreaLaw : MATLAB Function  TreatAsAtomicUnit=on
  EffectiveArea_m2 : Outport
  wires:
  BoundaryTP24/1 -> IdentifiedAreaLaw/1(boundaryTP24)
  IdentifiedAreaLaw/1(area) -> EffectiveArea_m2/1

== system Dll_Control_AFO_V8_5_R2019b/空气系统代理模型/G03_燃气涡轮二级进口/可压缩节流孔口 ==
  BoundaryTP24 : Inport  PortDimensions=24
  EffectiveArea_m2 : Inport  Port=2  PortDimensions=1
  GlobalParams7 : Inport  Port=3  PortDimensions=7
  ApplyMaximumFlow : MinMax  Inputs=2
  BoundRatio : Saturate  UpperLimit=1  LowerLimit=1e-6
  CriticalEnabled : Selector  InputPortWidth=7  IndexOptions=Index vector (dialog)  Indices=7  OutputSizes=1
  CriticalRatio : Fcn  Expr=(2/(u+1))^(u/(u-1))
  EnableForwardFlow : Switch  Criteria=u2 ~= 0
  ForwardFlow : RelationalOperator  Operator=>  OutDataTypeStr=boolean  RndMeth=Simplest
  Gamma : Selector  InputPortWidth=7  IndexOptions=Index vector (dialog)  Indices=4  OutputSizes=1
  GasR : Selector  InputPortWidth=7  IndexOptions=Index vector (dialog)  Indices=5  OutputSizes=1
  IsChoked : RelationalOperator  Operator=<=  OutDataTypeStr=boolean  RndMeth=Simplest
  MassFlowRaw : Product  Inputs=***/
  MuxGammaRatio : Mux  Inputs=2
  PhiChoked : Fcn  Expr=sqrt(u)*(2/(u+1))^((u+1)/(2*(u-1)))
  PhiSubcritical : Fcn  Expr=sqrt(2*u(1)/(u(1)-1)*(u(2)^(2/u(1))-u(2)^((u(1)+1)/u(1))))
  Pin_raw : Selector  InputPortWidth=24  IndexOptions=Index vector (dialog)  Indices=2*UpstreamBoundary  OutputSizes=1
  Pmin : Selector  InputPortWidth=7  IndexOptions=Index vector (dialog)  Indices=2  OutputSizes=1
  PoutPlusMinimumDrop : Sum
  Pout_raw : Selector  InputPortWidth=24  IndexOptions=Index vector (dialog)  Indices=2*DownstreamBoundary  OutputSizes=1
  PressureRatio : Product  Inputs=*/
  ProtectPin : MinMax  Function=max  Inputs=2
  ProtectPout : MinMax  Function=max  Inputs=2
  ProtectTin : MinMax  Function=max  Inputs=2
  RT : Product  Inputs=**
  SelectPhi : Switch  Criteria=u2 ~= 0
  SqrtRT : Math  Operator=sqrt  SignedPower=off  SaturateOnIntegerOverflow=on
  Tin_raw : Selector  InputPortWidth=24  IndexOptions=Index vector (dialog)  Indices=2*UpstreamBoundary-1  OutputSizes=1
  Tmin : Selector  InputPortWidth=7  IndexOptions=Index vector (dialog)  Indices=1  OutputSizes=1
  UseChokedBranch : Logic  AllPortsSameDT=off  OutDataTypeStr=boolean
  Wmax : Selector  InputPortWidth=7  IndexOptions=Index vector (dialog)  Indices=6  OutputSizes=1
  ZeroFlow : Constant  Value=0
  dPmin : Selector  InputPortWidth=7  IndexOptions=Index vector (dialog)  Indices=3  OutputSizes=1
  W_kgps : Outport
  wires:
  ApplyMaximumFlow/1 -> W_kgps/1
  Wmax/1 -> ApplyMaximumFlow/2
  EnableForwardFlow/1 -> ApplyMaximumFlow/1
  ZeroFlow/1 -> EnableForwardFlow/3
  ForwardFlow/1 -> EnableForwardFlow/2
  MassFlowRaw/1 -> EnableForwardFlow/1
  SqrtRT/1 -> MassFlowRaw/4
  EffectiveArea_m2/1 -> MassFlowRaw/3
  SelectPhi/1 -> MassFlowRaw/2
  RT/1 -> SqrtRT/1
  ProtectTin/1 -> RT/2
  GasR/1 -> RT/1
  PhiSubcritical/1 -> SelectPhi/3
  UseChokedBranch/1 -> SelectPhi/2
  PhiChoked/1 -> SelectPhi/1
  CriticalEnabled/1 -> UseChokedBranch/2
  IsChoked/1 -> UseChokedBranch/1
  CriticalRatio/1 -> IsChoked/2
  MuxGammaRatio/1 -> PhiSubcritical/1
  BoundRatio/1 -> IsChoked/1, MuxGammaRatio/2
  Gamma/1 -> MuxGammaRatio/1, PhiChoked/1, CriticalRatio/1
  PressureRatio/1 -> BoundRatio/1
  PoutPlusMinimumDrop/1 -> ForwardFlow/2
  ProtectPin/1 -> MassFlowRaw/1, PressureRatio/2, ForwardFlow/1
  dPmin/1 -> PoutPlusMinimumDrop/2
  ProtectPout/1 -> PressureRatio/1, PoutPlusMinimumDrop/1
  Pout_raw/1 -> ProtectPout/1
  Pmin/1 -> ProtectPout/2, ProtectPin/2
  Pin_raw/1 -> ProtectPin/1
  Tmin/1 -> ProtectTin/2
  Tin_raw/1 -> ProtectTin/1
  GlobalParams7/1 -> CriticalEnabled/1, Wmax/1, GasR/1, Gamma/1, dPmin/1, Pmin/1, Tmin/1
  BoundaryTP24/1 -> Pout_raw/1, Pin_raw/1, Tin_raw/1

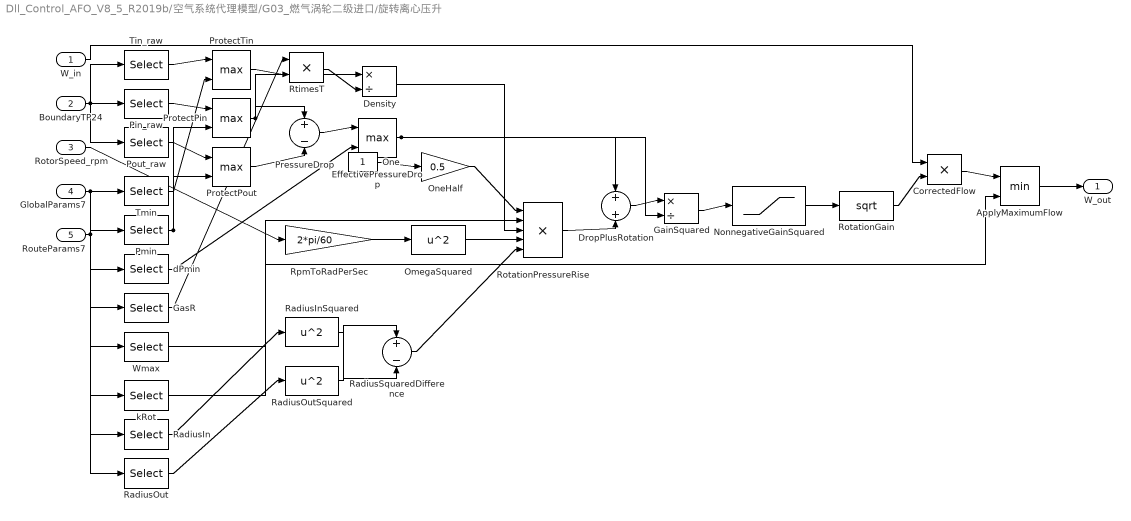
== system Dll_Control_AFO_V8_5_R2019b/空气系统代理模型/G03_燃气涡轮二级进口/旋转离心压升 ==
  W_in : Inport  PortDimensions=1
  BoundaryTP24 : Inport  Port=2  PortDimensions=24
  RotorSpeed_rpm : Inport  Port=3  PortDimensions=1
  GlobalParams7 : Inport  Port=4  PortDimensions=7
  RouteParams7 : Inport  Port=5  PortDimensions=7
  ApplyMaximumFlow : MinMax  Inputs=2
  CorrectedFlow : Product  Inputs=**
  Density : Product  Inputs=*/
  DropPlusRotation : Sum
  EffectivePressureDrop : MinMax  Function=max  Inputs=2
  GainSquared : Product  Inputs=*/
  GasR : Selector  InputPortWidth=7  IndexOptions=Index vector (dialog)  Indices=5  OutputSizes=1
  NonnegativeGainSquared : Saturate  UpperLimit=16  LowerLimit=0
  OmegaSquared : Math  Operator=square  SignedPower=off  SaturateOnIntegerOverflow=on
  One : Constant
  OneHalf : Gain  Gain=0.5
  Pin_raw : Selector  InputPortWidth=24  IndexOptions=Index vector (dialog)  Indices=2*UpstreamBoundary  OutputSizes=1
  Pmin : Selector  InputPortWidth=7  IndexOptions=Index vector (dialog)  Indices=2  OutputSizes=1
  Pout_raw : Selector  InputPortWidth=24  IndexOptions=Index vector (dialog)  Indices=2*DownstreamBoundary  OutputSizes=1
  PressureDrop : Sum  Inputs=+-
  ProtectPin : MinMax  Function=max  Inputs=2
  ProtectPout : MinMax  Function=max  Inputs=2
  ProtectTin : MinMax  Function=max  Inputs=2
  RadiusIn : Selector  InputPortWidth=7  IndexOptions=Index vector (dialog)  Indices=3  OutputSizes=1
  RadiusInSquared : Math  Operator=square  SignedPower=off  SaturateOnIntegerOverflow=on
  RadiusOut : Selector  InputPortWidth=7  IndexOptions=Index vector (dialog)  Indices=4  OutputSizes=1
  RadiusOutSquared : Math  Operator=square  SignedPower=off  SaturateOnIntegerOverflow=on
  RadiusSquaredDifference : Sum  Inputs=+-
  RotationGain : Math  Operator=sqrt  SignedPower=off  SaturateOnIntegerOverflow=on
  RotationPressureRise : Product  Inputs=*****
  RpmToRadPerSec : Gain  Gain=2*pi/60
  RtimesT : Product  Inputs=**
  Tin_raw : Selector  InputPortWidth=24  IndexOptions=Index vector (dialog)  Indices=2*UpstreamBoundary-1  OutputSizes=1
  Tmin : Selector  InputPortWidth=7  IndexOptions=Index vector (dialog)  Indices=1  OutputSizes=1
  Wmax : Selector  InputPortWidth=7  IndexOptions=Index vector (dialog)  Indices=6  OutputSizes=1
  dPmin : Selector  InputPortWidth=7  IndexOptions=Index vector (dialog)  Indices=3  OutputSizes=1
  kRot : Selector  InputPortWidth=7  IndexOptions=Index vector (dialog)  Indices=2  OutputSizes=1
  W_out : Outport
  wires:
  ApplyMaximumFlow/1 -> W_out/1
  Wmax/1 -> ApplyMaximumFlow/2
  CorrectedFlow/1 -> ApplyMaximumFlow/1
  RotationGain/1 -> CorrectedFlow/2
  W_in/1 -> CorrectedFlow/1
  NonnegativeGainSquared/1 -> RotationGain/1
  GainSquared/1 -> NonnegativeGainSquared/1
  DropPlusRotation/1 -> GainSquared/1
  RotationPressureRise/1 -> DropPlusRotation/2
  EffectivePressureDrop/1 -> GainSquared/2, DropPlusRotation/1
  dPmin/1 -> EffectivePressureDrop/2
  PressureDrop/1 -> EffectivePressureDrop/1
  ProtectPout/1 -> PressureDrop/2
  RadiusSquaredDifference/1 -> RotationPressureRise/5
  OmegaSquared/1 -> RotationPressureRise/4
  Density/1 -> RotationPressureRise/3
  kRot/1 -> RotationPressureRise/2
  OneHalf/1 -> RotationPressureRise/1
  One/1 -> OneHalf/1
  RadiusInSquared/1 -> RadiusSquaredDifference/2
  RadiusOutSquared/1 -> RadiusSquaredDifference/1
  RadiusOut/1 -> RadiusOutSquared/1
  RadiusIn/1 -> RadiusInSquared/1
  RpmToRadPerSec/1 -> OmegaSquared/1
  RotorSpeed_rpm/1 -> RpmToRadPerSec/1
  RtimesT/1 -> Density/2
  ProtectPin/1 -> PressureDrop/1, Density/1
  ProtectTin/1 -> RtimesT/2
  GasR/1 -> RtimesT/1
  Pout_raw/1 -> ProtectPout/1
  Pmin/1 -> ProtectPout/2, ProtectPin/2
  Pin_raw/1 -> ProtectPin/1
  Tmin/1 -> ProtectTin/2
  Tin_raw/1 -> ProtectTin/1
  RouteParams7/1 -> RadiusOut/1, RadiusIn/1, kRot/1
  GlobalParams7/1 -> Wmax/1, GasR/1, dPmin/1, Pmin/1, Tmin/1
  BoundaryTP24/1 -> Pout_raw/1, Pin_raw/1, Tin_raw/1

== system Dll_Control_AFO_V8_5_R2019b/空气系统代理模型/G03_燃气涡轮二级进口/流路可调参数 ==
  Mux_RouteParams7 : Mux  Inputs=7
  kRot : Constant  Value=0.5
  内半径_m : Constant  Value=0.052499999999999998
  初值流量_kgps : Constant  Value=0.165771616630528
  外半径_m : Constant  Value=0.053999999999999999
  时间常数_s : Constant  Value=0
  等效面积缩放 : Constant  Value=0.98686224740569006
  篦齿修正系数 : Constant
  RouteParams7 : Outport
  wires:
  等效面积缩放/1 -> Mux_RouteParams7/1
  kRot/1 -> Mux_RouteParams7/2
  内半径_m/1 -> Mux_RouteParams7/3
  外半径_m/1 -> Mux_RouteParams7/4
  时间常数_s/1 -> Mux_RouteParams7/5
  初值流量_kgps/1 -> Mux_RouteParams7/6
  篦齿修正系数/1 -> Mux_RouteParams7/7
  Mux_RouteParams7/1 -> RouteParams7/1

== system Dll_Control_AFO_V8_5_R2019b/空气系统代理模型/G03_燃气涡轮二级进口/盘腔热动态 ==
  W_in : Inport  PortDimensions=1
  RouteParams7 : Inport  Port=2  PortDimensions=7
  Alpha : Fcn  Expr=exp(-SampleTime_s/u)
  DynamicOrBypass : Switch  Criteria=u2 ~= 0
  One : Constant
  OneMinusAlpha : Sum  Inputs=+-
  ProtectTau : Saturate  UpperLimit=inf  LowerLimit=1e-9
  State : UnitDelay  InitialCondition=InitialFlowValue  SampleTime=SampleTime_s  HasFrameUpgradeWarning=on
  Tau_s : Selector  InputPortWidth=7  IndexOptions=Index vector (dialog)  Indices=5  OutputSizes=1
  Update : Sum
  UseBypass : simulink/Logic and Bit Operations/Compare To Constant  relop=<=  const=1e-12  OutDataTypeStr=boolean
  WeightedInput : Product  Inputs=**
  WeightedState : Product  Inputs=**
  W_out : Outport
  wires:
  DynamicOrBypass/1 -> W_out/1
  UseBypass/1 -> DynamicOrBypass/2
  Update/1 -> DynamicOrBypass/3, State/1
  WeightedState/1 -> Update/2
  WeightedInput/1 -> Update/1
  State/1 -> WeightedState/1
  OneMinusAlpha/1 -> WeightedInput/2
  W_in/1 -> DynamicOrBypass/1, WeightedInput/1
  Alpha/1 -> WeightedState/2, OneMinusAlpha/2
  One/1 -> OneMinusAlpha/1
  ProtectTau/1 -> Alpha/1
  Tau_s/1 -> UseBypass/1, ProtectTau/1
  RouteParams7/1 -> Tau_s/1

== system Dll_Control_AFO_V8_5_R2019b/空气系统代理模型/G03_燃气涡轮二级进口/辨识等效面积 ==
  BoundaryTP24 : Inport  PortDimensions=24
  IdentifiedAreaLaw : MATLAB Function  TreatAsAtomicUnit=on
  EffectiveArea_m2 : Outport
  wires:
  BoundaryTP24/1 -> IdentifiedAreaLaw/1(boundaryTP24)
  IdentifiedAreaLaw/1(area) -> EffectiveArea_m2/1

== system Dll_Control_AFO_V8_5_R2019b/空气系统代理模型/G04_燃气涡轮二级出口/可压缩节流孔口 ==
  BoundaryTP24 : Inport  PortDimensions=24
  EffectiveArea_m2 : Inport  Port=2  PortDimensions=1
  GlobalParams7 : Inport  Port=3  PortDimensions=7
  ApplyMaximumFlow : MinMax  Inputs=2
  BoundRatio : Saturate  UpperLimit=1  LowerLimit=1e-6
  CriticalEnabled : Selector  InputPortWidth=7  IndexOptions=Index vector (dialog)  Indices=7  OutputSizes=1
  CriticalRatio : Fcn  Expr=(2/(u+1))^(u/(u-1))
  EnableForwardFlow : Switch  Criteria=u2 ~= 0
  ForwardFlow : RelationalOperator  Operator=>  OutDataTypeStr=boolean  RndMeth=Simplest
  Gamma : Selector  InputPortWidth=7  IndexOptions=Index vector (dialog)  Indices=4  OutputSizes=1
  GasR : Selector  InputPortWidth=7  IndexOptions=Index vector (dialog)  Indices=5  OutputSizes=1
  IsChoked : RelationalOperator  Operator=<=  OutDataTypeStr=boolean  RndMeth=Simplest
  MassFlowRaw : Product  Inputs=***/
  MuxGammaRatio : Mux  Inputs=2
  PhiChoked : Fcn  Expr=sqrt(u)*(2/(u+1))^((u+1)/(2*(u-1)))
  PhiSubcritical : Fcn  Expr=sqrt(2*u(1)/(u(1)-1)*(u(2)^(2/u(1))-u(2)^((u(1)+1)/u(1))))
  Pin_raw : Selector  InputPortWidth=24  IndexOptions=Index vector (dialog)  Indices=2*UpstreamBoundary  OutputSizes=1
  Pmin : Selector  InputPortWidth=7  IndexOptions=Index vector (dialog)  Indices=2  OutputSizes=1
  PoutPlusMinimumDrop : Sum
  Pout_raw : Selector  InputPortWidth=24  IndexOptions=Index vector (dialog)  Indices=2*DownstreamBoundary  OutputSizes=1
  PressureRatio : Product  Inputs=*/
  ProtectPin : MinMax  Function=max  Inputs=2
  ProtectPout : MinMax  Function=max  Inputs=2
  ProtectTin : MinMax  Function=max  Inputs=2
  RT : Product  Inputs=**
  SelectPhi : Switch  Criteria=u2 ~= 0
  SqrtRT : Math  Operator=sqrt  SignedPower=off  SaturateOnIntegerOverflow=on
  Tin_raw : Selector  InputPortWidth=24  IndexOptions=Index vector (dialog)  Indices=2*UpstreamBoundary-1  OutputSizes=1
  Tmin : Selector  InputPortWidth=7  IndexOptions=Index vector (dialog)  Indices=1  OutputSizes=1
  UseChokedBranch : Logic  AllPortsSameDT=off  OutDataTypeStr=boolean
  Wmax : Selector  InputPortWidth=7  IndexOptions=Index vector (dialog)  Indices=6  OutputSizes=1
  ZeroFlow : Constant  Value=0
  dPmin : Selector  InputPortWidth=7  IndexOptions=Index vector (dialog)  Indices=3  OutputSizes=1
  W_kgps : Outport
  wires:
  ApplyMaximumFlow/1 -> W_kgps/1
  Wmax/1 -> ApplyMaximumFlow/2
  EnableForwardFlow/1 -> ApplyMaximumFlow/1
  ZeroFlow/1 -> EnableForwardFlow/3
  ForwardFlow/1 -> EnableForwardFlow/2
  MassFlowRaw/1 -> EnableForwardFlow/1
  SqrtRT/1 -> MassFlowRaw/4
  EffectiveArea_m2/1 -> MassFlowRaw/3
  SelectPhi/1 -> MassFlowRaw/2
  RT/1 -> SqrtRT/1
  ProtectTin/1 -> RT/2
  GasR/1 -> RT/1
  PhiSubcritical/1 -> SelectPhi/3
  UseChokedBranch/1 -> SelectPhi/2
  PhiChoked/1 -> SelectPhi/1
  CriticalEnabled/1 -> UseChokedBranch/2
  IsChoked/1 -> UseChokedBranch/1
  CriticalRatio/1 -> IsChoked/2
  MuxGammaRatio/1 -> PhiSubcritical/1
  BoundRatio/1 -> IsChoked/1, MuxGammaRatio/2
  Gamma/1 -> MuxGammaRatio/1, PhiChoked/1, CriticalRatio/1
  PressureRatio/1 -> BoundRatio/1
  PoutPlusMinimumDrop/1 -> ForwardFlow/2
  ProtectPin/1 -> MassFlowRaw/1, PressureRatio/2, ForwardFlow/1
  dPmin/1 -> PoutPlusMinimumDrop/2
  ProtectPout/1 -> PressureRatio/1, PoutPlusMinimumDrop/1
  Pout_raw/1 -> ProtectPout/1
  Pmin/1 -> ProtectPout/2, ProtectPin/2
  Pin_raw/1 -> ProtectPin/1
  Tmin/1 -> ProtectTin/2
  Tin_raw/1 -> ProtectTin/1
  GlobalParams7/1 -> CriticalEnabled/1, Wmax/1, GasR/1, Gamma/1, dPmin/1, Pmin/1, Tmin/1
  BoundaryTP24/1 -> Pout_raw/1, Pin_raw/1, Tin_raw/1
